simulink model "Analog Programmable Electronic Load - Simulink"  (R2022b)
settings: Solver=VariableStepAuto  StartTime=0.0  StopTime=0.1  RelTol=1e-3
libraries: fl_lib x12, ee_lib x5, nesl_utility x5
settings Model: Creator=gobis  LastModifiedBy=gobis

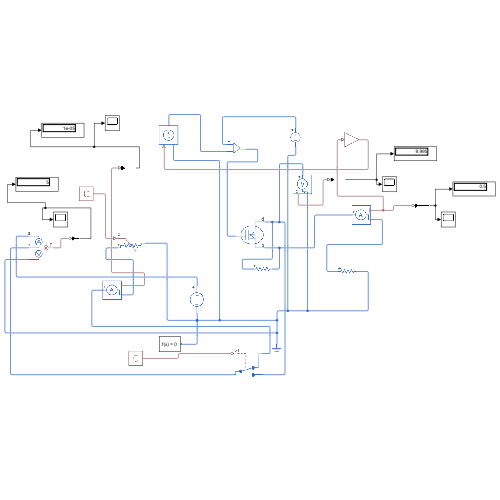
[thumbnail: Simulink's stored preview of the top-level diagram]
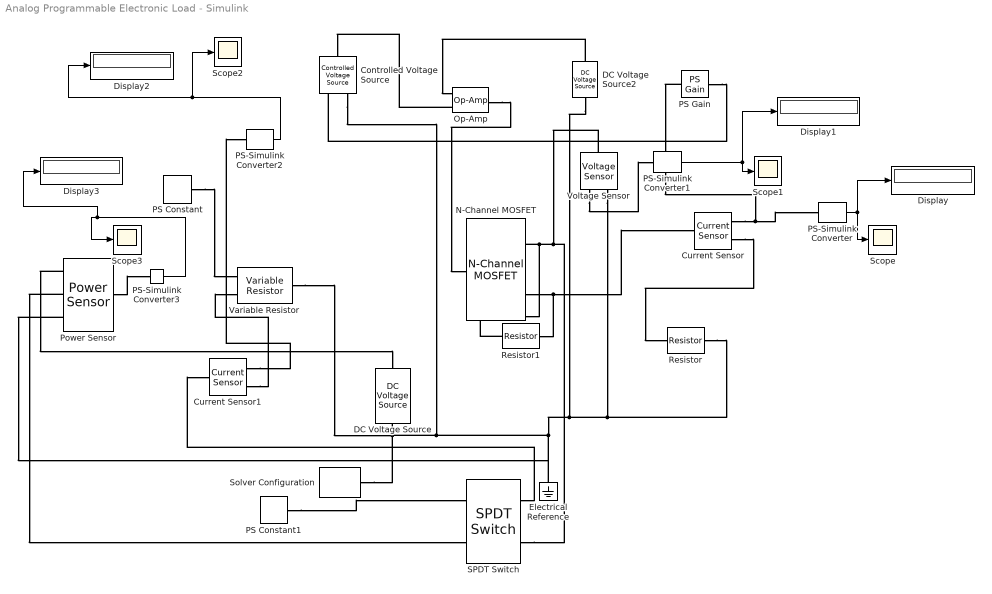
== system Analog Programmable Electronic Load - Simulink ==
  Controlled Voltage Source : fl_lib/Electrical/Electrical Sources/Controlled Voltage Source
  Current Sensor : fl_lib/Electrical/Electrical Sensors/Current Sensor
  Current Sensor1 : fl_lib/Electrical/Electrical Sensors/Current Sensor
  DC Voltage Source : ee_lib/Additional Components/SPICE Sources/DC Voltage Source  DC=10 V
  DC Voltage Source2 : ee_lib/Additional Components/SPICE Sources/DC Voltage Source  DC=0.5 V
  Display{,1..3} (4 alike) : Display
  Electrical Reference : fl_lib/Electrical/Electrical Elements/Electrical Reference
  N-Channel MOSFET : ee_lib/Semiconductors & Converters/N-Channel MOSFET  paramTerminal=ee.enum.mosfet.numberOfTerminals.three  parameterization=ee.enum.mosfet.parameterization.datasheet  Beta=5.0 A/V^2  Rds=0.025 Ohm  Id=6.0 A  Vgs=10 V  Vth=1.7 V  Vth0=1.7 V  lam=0 1/V  gamma_vth=0.5 V^(1/2)  phib=0.5 V  Vth1=1.9071 V  Vbs1=-1 V  Vth2=2.066 V  Vbs2=-2 V  Tmeas=25 degC  Vgs_vec=[-.5, 2, 3, 4, 5] V  Vds_vec=[0, 2, 4, 8, 12, 16, 20] V  Vbs_vec=[0, -4, -6, -12] V  T_vec=[25, 125] degC  Vth_vec=[.4, 1.2, 1.4, 1.45] V  Vth_mat=[.4, .35; 1.2, 1.15; 1.4, 1.35; 1.45, 1.4] V  Ids_mat=[0, 0, 0, 0, 0, 0, 0; 0, .003, .0038, .0043, .0046, .0048, .0049; 0, .0055, .008, .009, .0095, .01, .0101; 0, .0115, .016, .018, .019, .0195, .02; 0, .0152, .0225, .0265, .028, .0295, .03] A  Ids_mat0=[0, 0, 0, 0, 0, 0, 0; 0, .003, .0038, .0043, .0046, .0048, .0049; 0, .0055, .008, .009, .0095, .01, .0101; 0, .0115, .016, .018, .019, .0195, .02; 0, .0152, .0225, .0265, .028, .0295, .03] A  Ids_mat_3D=zeros(5, 7, 2) A  Ids_mat_3D0=zeros(5, 7, 2) A  IV_table_symmetry=ee.enum.mosfet.symmetricNIV.no  RS=0.0001 Ohm  RD=0.01 Ohm  RB=0.001 Ohm  C_param=ee.enum.mosfet.capacitanceParam.fixedciss  C_GS=270 pF  C_GD=80 pF  C_GB=0 pF  C_DS=0 pF  C_iss=350 pF  C_rss=80 pF  C_oss=0 pF  C_iss_vec=[720, 700, 590, 470, 390, 310] pF  C_rss_vec=[450, 400, 300, 190, 95, 55] pF  C_oss_vec=[900, 810, 690, 420, 270, 170] pF  C_GS_vec=[270, 300, 290, 280, 295, 255] pF  C_GD_vec=[450, 400, 300, 190, 95, 55] pF  C_GB_vec=[270, 300, 290, 280, 295, 255] pF  C_Vgs_vec=0 V  C_DS_vec=[450, 410, 390, 230, 175, 115] pF  C_Vds_vec=[.1, .3, 1, 3, 10, 30] V  V_GS_for_cap_data=0 V  charge_linearity_param=ee.enum.mosfet.cgdLinearity.constant  C_OX=200 pF  V_C_OX=-0.5 V  charge_linearity_param_vgb=ee.enum.mosfet.cgbLinearity.instantly  charge_linearity_param_with_vgb=ee.enum.mosfet.cgbLinearityWithSeparateCgb.instantly  Di_param=ee.enum.mosfet.diodeParam.no  IsDiode=1e-12 A  Vbi=0.6 V  n=1  Cj0Diode=0 pF  TT=50e-9 s  Tmeas_dio=25 degC  TableTypeNoT=ee.enum.mosfet.tableType.IfMat  TableType=ee.enum.diode.tableType.IfMat  IfVec=[.07, .12, .19, 1.75, 4.24, 7.32, 11.2] A  IfMat=[.07, .12, .19, 1.75, 4.24, 7.32, 11.2; .16, .3, .72, 2.14, 4.02, 6.35, 9.12] A  VfVecV=[.9, 1.15, 1.25, 1.5, 1.75, 2.17, 2.6, 2.85] V  VfMatV=[.9, 1.15, 1.25, 1.5, 1.75, 2.17, 2.6, 2.85; .58, .68, .75, 1.1, 1.38, 1.77, 2.27, 2.7] V  TjVec=[25, 125] degC  VfVec=[.5, .7, .9, 1.3, 1.7, 2.1, 2.5] V  IfVecV=[.1, .2, .5, 1, 2, 4, 7, 10] A  prmDatasheet=ee.enum.temperatureParameterization.none  prmEquCoeff=ee.enum.temperatureParameterization.none  dVth_dT=-6 mV/K  dVth0_dT=-6 mV/K  Rds_T2=0.037 Ohm  BEXDatasheet=-1.5  BEXEquCoeff=-1.5  etaisDatasheet=3  etaisEquCoeff=3  Tmeas2=125 degC  etaisTabulated=3  TdeviceDatasheet=25 degC  TdeviceEquCoeff=25 degC  TdeviceTabulated=25 degC  enable_faults=simscape.enum.onoff.off  fault_trigger=ee.enum.faults.faultTrigger.temporal  t_fault=inf s  max_permissible_Vgs=inf V  max_permissible_Vds=inf V  max_permissible_Vdb=inf V  max_permissible_Ids=inf A  t_fail_on_Ids=1 s  max_permissible_Idiode=inf A  t_fail_on_Idiode=1 s  max_permissible_dVdt=inf V/s  tau_fault=1e-3 s  fault_types=ee.enum.mosfet.faults.open  fault_types_4T=ee.enum.mosfet.faultsFourTerminals.open  RG_open=1e6 Ohm  RD_open=1000 Ohm  RS_open=1000 Ohm  RB_open=1000 Ohm  GDS_short=1000 1/Ohm  GDB_short=1000 1/Ohm  GSB_short=1000 1/Ohm  location_GOS=0  G_GOS=1000 1/Ohm  D_GOS=ee.enum.include.no  Is_GOS=0 A  Vbi_GOS=0.6 V  n_GOS=1  Cj0_GOS=0 pF  TT_GOS=50e-9 s  Beta_scale=100  dVth_faulted=0 V  lam_faulted=0 1/V  gamma_scale=100  dPhib_faulted=0 V  Vgs_vec_faulted=[-.5, 2, 3, 4, 5] V  Vds_vec_faulted=[0, 2, 4, 8, 12, 16, 20] V  Vbs_vec_faulted=[0, -4, -6, -12] V  Vth_vec_faulted=[.4, 1.2, 1.4, 1.45] V  Vth_mat_faulted=[.4, .35; 1.2, 1.15; 1.4, 1.35; 1.45, 1.4] V  Ids_mat_faulted=[0, 0, 0, 0, 0, 0, 0; 0, .003, .0038, .0043, .0046, .0048, .0049; 0, .0055, .008, .009, .0095, .01, .0101; 0, .0115, .016, .018, .019, .0195, .02; 0, .0152, .0225, .0265, .028, .0295, .03] A  Ids_mat0_faulted=[0, 0, 0, 0, 0, 0, 0; 0, .003, .0038, .0043, .0046, .0048, .0049; 0, .0055, .008, .009, .0095, .01, .0101; 0, .0115, .016, .018, .019, .0195, .02; 0, .0152, .0225, .0265, .028, .0295, .03] A  Ids_mat_3D_faulted=zeros(5, 7, 2) A  Ids_mat_3D0_faulted=zeros(5, 7, 2) A  RS_faulted=0.0001 Ohm  RD_faulted=0.01 Ohm  RB_faulted=0.001 Ohm  IsDiode_faulted=0 A  Vbi_faulted=0.6 V  n_faulted=1  Cj0Diode_scale=100  TT_faulted=50e-9 s  IfVec_faulted=[.07, .12, .19, 1.75, 4.24, 7.32, 11.2] A  IfMat_faulted=[.07, .12, .19, 1.75, 4.24, 7.32, 11.2; .16, .3, .72, 2.14, 4.02, 6.35, 9.12] A  VfVecV_faulted=[.9, 1.15, 1.25, 1.5, 1.75, 2.17, 2.6, 2.85] V  VfMatV_faulted=[.9, 1.15, 1.25, 1.5, 1.75, 2.17, 2.6, 2.85; .58, .68, .75, 1.1, 1.38, 1.77, 2.27, 2.7] V  VfVec_faulted=[.5, .7, .9, 1.3, 1.7, 2.1, 2.5] V  IfVecV_faulted=[.1, .2, .5, 1, 2, 4, 7, 10] A  C_GS_scale=100  C_GD_scale=100  C_GB_scale=100  C_DS_scale=100  C_OX_scale=100  V_C_OX_faulted=-0.5 V  C_iss_vec_faulted=[720, 700, 590, 470, 390, 310] pF  C_rss_vec_faulted=[450, 400, 300, 190, 95, 55] pF  C_oss_vec_faulted=[900, 810, 690, 420, 270, 170] pF  C_GS_vec_faulted=[270, 300, 290, 280, 295, 255] pF  C_GD_vec_faulted=[450, 400, 300, 190, 95, 55] pF  C_GB_vec_faulted=[270, 300, 290, 280, 295, 255] pF  C_Vgs_vec_faulted=0 V  C_DS_vec_faulted=[450, 410, 390, 230, 175, 115] pF  C_Vds_vec_faulted=[.1, .3, 1, 3, 10, 30] V  V_GS_for_cap_data_faulted=0 V  i_g_specify=off  i_g_priority=None  i_g=0 A  i_g_nominal_specify=off  i_g_nominal_unit=A  i_g_nominal_value=1  i_d_specify=off  i_d_priority=None  i_d=0 A  i_d_nominal_specify=off  i_d_nominal_unit=A  i_d_nominal_value=1  i_b_specify=off  i_b_priority=None  i_b=0 A  i_b_nominal_specify=off  i_b_nominal_unit=A  i_b_nominal_value=1  voltage_gs_specify=off  voltage_gs_priority=None  voltage_gs=0 V  voltage_gs_nominal_specify=off  voltage_gs_nominal_unit=V  voltage_gs_nominal_value=1  voltage_ds_specify=off  voltage_ds_priority=None  voltage_ds=0 V  voltage_ds_nominal_specify=off  voltage_ds_nominal_unit=V  voltage_ds_nominal_value=1  voltage_bs_specify=off  voltage_bs_priority=None  voltage_bs=0 V  voltage_bs_nominal_specify=off  voltage_bs_nominal_unit=V  voltage_bs_nominal_value=1  v_Cgs_specify=off  v_Cgs_priority=High  v_Cgs=0 V  v_Cgs_nominal_specify=off  v_Cgs_nominal_unit=V  v_Cgs_nominal_value=1  v_Cds_specify=off  v_Cds_priority=High  v_Cds=0 V  v_Cds_nominal_specify=off  v_Cds_nominal_unit=V  v_Cds_nominal_value=1  v_Cbs_specify=off  v_Cbs_priority=High  v_Cbs=0 V  v_Cbs_nominal_specify=off  v_Cbs_nominal_unit=V  v_Cbs_nominal_value=1  thermal_network_parameterization=ee.enum.thermalNetworkTopology.junctionCase  Rth=[0, 10] K/W  Rth_Cauer=[1, 3, 10] K/W  Rth_Foster=[4, 6] K/W  thermal_mass_parameterization=ee.enum.thermalNetwork.timeconstant  thermal_mass=[0, 1] J/K  thermal_mass_Cauer=[.1, .3, 1] J/K  thermal_mass_Foster=[1.5, 3] J/K  thermal_time_constant=[0, 10] s  thermal_time_constant_Cauer=[1, 3, 10] s  thermal_time_constant_Foster=[6, 18] s  thermal_mass_initial_temperatures=[25, 25] degC  thermal_mass_initial_temperatures_Cauer=[25, 25, 25] degC  Tvec_initial_Foster=[25, 25, 25, 25] degC  max_permissible_temperature=inf K  t_fail_on_temperature=1 s  betaref=18 A/V^2  Vfbref=-1.1 V  gamma=3.5 V^(1/2)  phib2ref=1 V  thesatref=0.4 1/V  alpha=0  Vp=5e-2 V  thesrref=0 1/V  m=8  Tref=25 degC  Rsref=2e-3 Ohm  Rdref=0.17 Ohm  Rgref=8.4 Ohm  Rbref=2e-3 Ohm  Cox=1500 pF  Cgso=100 pF  Cgdo=14 pF  Isref=5.2e-13 A  Cj0=480 pF  Tprm=1  etabet=1.3  Stvfb=5e-4 V/K  Stphib=-8.5e-4 V/K  etasat=1.04  etasr=0.65  etar=0.95  etais=3  Tsim=25 degC  Ig_specify=off  Ig_priority=None  Ig=0 A  Ig_nominal_specify=off  Ig_nominal_unit=A  Ig_nominal_value=1  Ids_specify=off  Ids_priority=None  Ids=0 A  Ids_nominal_specify=off  Ids_nominal_unit=A  Ids_nominal_value=1  Ib_specify=off  Ib_priority=None  Ib=0 A  Ib_nominal_specify=off  Ib_nominal_unit=A  Ib_nominal_value=1  V_gs_specify=off  V_gs_priority=None  V_gs=0 V  V_gs_nominal_specify=off  V_gs_nominal_unit=V  V_gs_nominal_value=1  V_ds_specify=off  V_ds_priority=None  V_ds=0 V  V_ds_nominal_specify=off  V_ds_nominal_unit=V  V_ds_nominal_value=1  V_bs_specify=off  V_bs_priority=None  V_bs=0 V  V_bs_nominal_specify=off  V_bs_nominal_unit=V  V_bs_nominal_value=1  QGoverCox_specify=off  QGoverCox_priority=None  QGoverCox=0 V  QGoverCox_nominal_specify=off  QGoverCox_nominal_unit=V  QGoverCox_nominal_value=1  QDoverCox_specify=off  QDoverCox_priority=None  QDoverCox=0 V  QDoverCox_nominal_specify=off  QDoverCox_nominal_unit=V  QDoverCox_nominal_value=1  QBoverCox_specify=off  QBoverCox_priority=None  QBoverCox=0 V  QBoverCox_nominal_specify=off  QBoverCox_nominal_unit=V  QBoverCox_nominal_value=1  T0=[25, 25] degC  T0_Cauer=[25, 25, 25] degC
  Op-Amp : fl_lib/Electrical/Electrical Elements/Op-Amp  outI_specify=off  outI_priority=None  outI=0 A  outI_nominal_specify=off  outI_nominal_unit=A  outI_nominal_value=1
  PS Constant : fl_lib/Physical Signals/Sources/PS Constant  constant=20 V/A
  PS Constant1 : fl_lib/Physical Signals/Sources/PS Constant  constant=1 V
  PS Gain : fl_lib/Physical Signals/Functions/PS Gain  gain=1 V/A
  PS-Simulink Converter{,1..3} (4 alike) : nesl_utility/PS-Simulink Converter  PhysicalDomain=network_engine_domain  SubClassName=ps_output  LeftPortType=input  RightPortType=output  PseudoPeriodic=off  Frequencies=[]  VectorFormat=inherit  Unit=inherit  AffineConversion=off
  Power Sensor : ee_lib/Sensors & Transducers/Power Sensor  measurement_type=1  averaging_period=1e-4 s
  Resistor : fl_lib/Electrical/Electrical Elements/Resistor  R=10 Ohm  i_specify=off  i_priority=None  i=0 A  i_nominal_specify=off  i_nominal_unit=A  i_nominal_value=1  v_specify=off  v_priority=None  v=0 V  v_nominal_specify=off  v_nominal_unit=V  v_nominal_value=1
  Resistor1 : fl_lib/Electrical/Electrical Elements/Resistor  R=1000000 Ohm  i_specify=off  i_priority=None  i=0 A  i_nominal_specify=off  i_nominal_unit=A  i_nominal_value=1  v_specify=off  v_priority=None  v=0 V  v_nominal_specify=off  v_nominal_unit=V  v_nominal_value=1
  SPDT Switch : ee_lib/Switches & Breakers/SPDT Switch  R_closed=0.01 Ohm  G_open=1e-6 S  Threshold=0.5 V  Width=0 V  model_dynamics=0  t_on=1e-3 s  t_off=1e-3 s  initial_vT=0 V
  Scope{,1..3} (4 alike) : Scope
  Solver Configuration : nesl_utility/Solver Configuration  PhysicalDomain=network_engine_domain  SubClassName=solver  LeftPortType=input  RightPortType=generic  Tones=[]  Harmonics=[]  SimulateNoise=off  Profile=off  UseLocalSampling=off  EnableSwitchedLinearOptims=on  FrequencyDomain=off  UseCCode=off  RelTol=0.001  AbsTol=0.001  MinStep=1e-09  ToWorkspace=off  RevertToSquareIcSolve=off  NumHomotopyIterations=100  PhasorMode=off  PhasorModeNumHarmonics=1  ConsistencySolver=NEWTON_XTOL_AFTER_FTOL  IndexReductionMethod=DerivativeReplacement  DoDC=off  ResidualTolerance=1e-09  ConsistencyTolSource=GLOBAL  ConsistencyAbsTol=0.001  ConsistencyRelTol=0.001  ConsistencyTolFactor=0.001  UseLocalSolver=off  LocalSolverChoice=NE_BACKWARD_EULER_ADVANCER  ResolveIndetEquations=on  FunctionEvalNumThread=1  LocalSolverSampleTime=0.001  DoFixedCost=off  MaxNonlinIter=3  MaxModeIter=2  ComputeImpulses=off  ImpulseIterations=2  LinearAlgebra=auto  LinearAlgebraNumThread=0  EquationFormulation=NE_TIME_EF  DelaysMemoryBudget=1024  AutomaticFiltering=on  FilteringTimeConstant=0.001  PartitionStorageMethod=AS_NEEDED  PartitionMemoryBudget=1024  PartitionMethod=ROBUST
  Variable Resistor : fl_lib/Electrical/Electrical Elements/Variable Resistor  Rmin=1 Ohm  i_specify=off  i_priority=None  i=0 A  i_nominal_specify=off  i_nominal_unit=A  i_nominal_value=1  v_specify=off  v_priority=None  v=0 V  v_nominal_specify=off  v_nominal_unit=V  v_nominal_value=1
  Voltage Sensor : fl_lib/Electrical/Electrical Sensors/Voltage Sensor
  wires:
  PS-Simulink Converter2/1 -> Display2/1, Scope2/1
  PS-Simulink Converter1/1 -> Display1/1, Scope1/1
  PS-Simulink Converter/1 -> Display/1, Scope/1
  PS-Simulink Converter3/1 -> Display3/1, Scope3/1
  connections:
  Resistor/RConn1 -- Voltage Sensor/RConn2 -- Electrical Reference/LConn1 -- Power Sensor/LConn3 -- Controlled Voltage Source/RConn2 -- Solver Configuration/RConn1 -- DC Voltage Source/RConn1 -- Variable Resistor/RConn1 -- DC Voltage Source2/RConn1
  Voltage Sensor/RConn1 -- PS-Simulink Converter1/LConn1
  Current Sensor/RConn1 -- PS Gain/LConn1 -- PS-Simulink Converter/LConn1
  Op-Amp/LConn2 -- Controlled Voltage Source/LConn1
  Current Sensor1/RConn2 -- Variable Resistor/LConn2
  PS Constant/RConn1 -- Variable Resistor/LConn1
  Current Sensor/RConn2 -- Resistor/LConn1
  N-Channel MOSFET/RConn2 -- Resistor1/RConn1 -- Current Sensor/LConn1
  Current Sensor1/RConn1 -- PS-Simulink Converter2/LConn1
  DC Voltage Source2/LConn1 -- Op-Amp/LConn1
  Op-Amp/RConn1 -- N-Channel MOSFET/LConn1
  PS Gain/RConn1 -- Controlled Voltage Source/RConn1
  Voltage Sensor/LConn1 -- Resistor1/LConn1 -- N-Channel MOSFET/RConn1 -- SPDT Switch/RConn2
  Power Sensor/LConn1 -- DC Voltage Source/LConn1
  PS Constant1/RConn1 -- SPDT Switch/LConn1
  SPDT Switch/RConn1 -- Current Sensor1/LConn1
  Power Sensor/LConn2 -- SPDT Switch/LConn2
  Power Sensor/RConn1 -- PS-Simulink Converter3/LConn1
